simulink model "gnc_GlobalReplanner"  (R2026b)
settings: Solver=VariableStepAuto
values from neighbouring files (symbols this model uses):
  Ts = prm.Ts    [gnc_missionFSM.m]    (also in gnc_mpcPlantUpdate.m)
undefined symbols (not defined in the file or in its folder): P
settings Model: Creator=aomar  LastModifiedBy=aomar

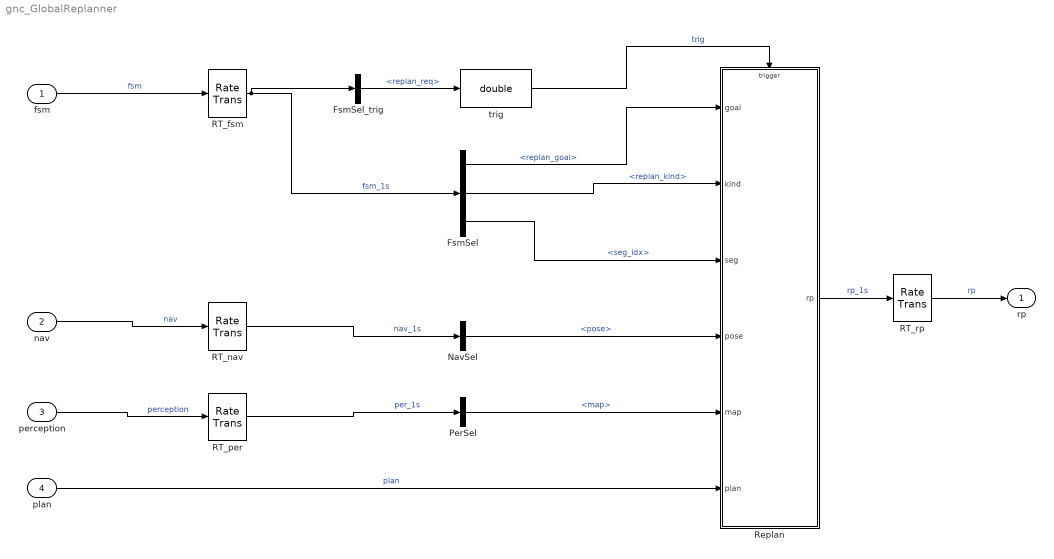
== system gnc_GlobalReplanner ==
  fsm : Inport  OutDataTypeStr=Bus: Bus_FsmOut  SampleTime=Ts.gnc
  nav : Inport  Port=2  OutDataTypeStr=Bus: Bus_NavCond  SampleTime=Ts.gnc
  perception : Inport  Port=3  OutDataTypeStr=Bus: Bus_Perception  SampleTime=Ts.perception
  plan : Inport  Port=4  OutDataTypeStr=Bus: Bus_MissionPlan
  FsmSel : BusSelector  OutputSignals=replan_goal,replan_kind,seg_idx
  FsmSel_trig : BusSelector  OutputSignals=replan_req
  NavSel : BusSelector  OutputSignals=pose
  PerSel : BusSelector  OutputSignals=map
  RT_fsm : RateTransition  OutPortSampleTime=Ts.plan
  RT_nav : RateTransition  OutPortSampleTime=Ts.plan
  RT_per : RateTransition  OutPortSampleTime=Ts.plan
  RT_rp : RateTransition  OutPortSampleTime=Ts.gnc
  Replan : Subsystem  TreatAsAtomicUnit=on
  trig : DataTypeConversion  OutDataTypeStr=double  RndMeth=Nearest
  rp : Outport  OutDataTypeStr=Bus: Bus_ReplanResult
  wires:
  fsm/1 -> RT_fsm/1  "fsm"
  nav/1 -> RT_nav/1  "nav"
  perception/1 -> RT_per/1  "perception"
  plan/1 -> Replan/6(plan)  "plan"
  RT_fsm/1 -> FsmSel/1, FsmSel_trig/1  "fsm_1s"
  RT_nav/1 -> NavSel/1  "nav_1s"
  RT_per/1 -> PerSel/1  "per_1s"
  FsmSel_trig/1 -> trig/1  "<replan_req>"
  FsmSel/1 -> Replan/1(goal)  "<replan_goal>"
  FsmSel/2 -> Replan/2(kind)  "<replan_kind>"
  FsmSel/3 -> Replan/3(seg)  "<seg_idx>"
  NavSel/1 -> Replan/4(pose)  "<pose>"
  PerSel/1 -> Replan/5(map)  "<map>"
  trig/1 -> Replan/Trigger  "trig"
  Replan/1(rp) -> RT_rp/1  "rp_1s"
  RT_rp/1 -> rp/1  "rp"

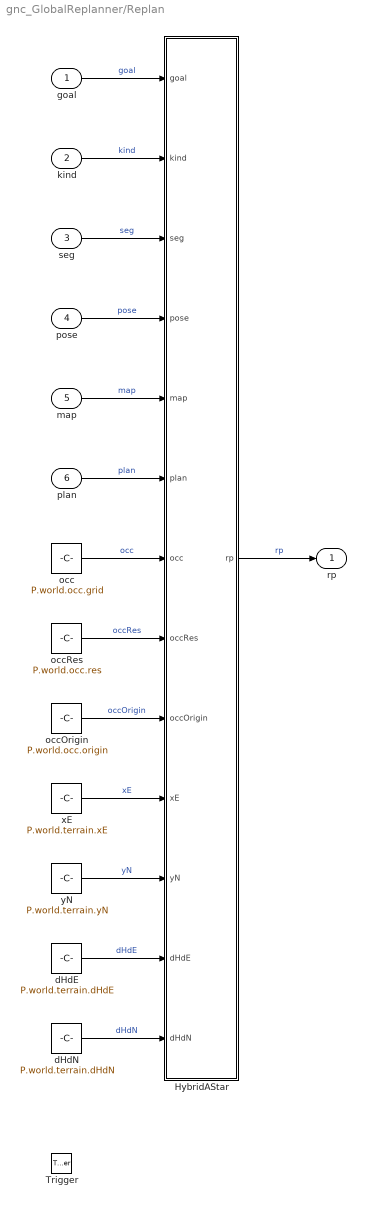
== system gnc_GlobalReplanner/Replan ==
  goal : Inport
  kind : Inport  Port=2
  seg : Inport  Port=3
  pose : Inport  Port=4
  map : Inport  Port=5
  plan : Inport  Port=6
  Trigger : TriggerPort  TriggerType=either  VariantControl=(inherit)  InitialTriggerSignalState=zero  PortDimensions=1
  HybridAStar : MATLAB Function  TreatAsAtomicUnit=on  mask{prm=P.gnc.hastar}
  dHdE : Constant  Value=P.world.terrain.dHdE  OutDataTypeStr=double
  dHdN : Constant  Value=P.world.terrain.dHdN  OutDataTypeStr=double
  occ : Constant  Value=P.world.occ.grid  OutDataTypeStr=boolean
  occOrigin : Constant  Value=P.world.occ.origin  OutDataTypeStr=double
  occRes : Constant  Value=P.world.occ.res  OutDataTypeStr=double
  xE : Constant  Value=P.world.terrain.xE  OutDataTypeStr=double
  yN : Constant  Value=P.world.terrain.yN  OutDataTypeStr=double
  rp : Outport  OutDataTypeStr=Bus: Bus_ReplanResult  InitialOutput=P.ic.Bus_ReplanResult
  wires:
  goal/1 -> HybridAStar/1(goal)  "goal"
  kind/1 -> HybridAStar/2(kind)  "kind"
  seg/1 -> HybridAStar/3(seg)  "seg"
  pose/1 -> HybridAStar/4(pose)  "pose"
  map/1 -> HybridAStar/5(map)  "map"
  plan/1 -> HybridAStar/6(plan)  "plan"
  occ/1 -> HybridAStar/7(occ)  "occ"
  occRes/1 -> HybridAStar/8(occRes)  "occRes"
  occOrigin/1 -> HybridAStar/9(occOrigin)  "occOrigin"
  xE/1 -> HybridAStar/10(xE)  "xE"
  yN/1 -> HybridAStar/11(yN)  "yN"
  dHdE/1 -> HybridAStar/12(dHdE)  "dHdE"
  dHdN/1 -> HybridAStar/13(dHdN)  "dHdN"
  HybridAStar/1(rp) -> rp/1  "rp"

== matlab function gnc_GlobalReplanner/Replan/HybridAStar ==
  settings: description=Hybrid A* replanning (gnc spec 4.4); body subsystems/gnc/gnc_globalReplanner.m.
  data: goal input; rp output Bus: Bus_ReplanResult; kind input; seg input; pose input; map input Bus: Bus_TebMapInfo; plan input Bus: Bus_MissionPlan; occ input; occRes input; occOrigin input; xE input; yN input; dHdE input; dHdN input; prm parameter
function rp = fcn(goal, kind, seg, pose, map, plan, occ, occRes, occOrigin, xE, yN, dHdE, dHdN, prm)
%#codegen
rp = gnc_globalReplanner(goal, kind, seg, pose, map, plan, occ, occRes, occOrigin, ...
    struct('xE', xE, 'yN', yN, 'dHdE', dHdE, 'dHdN', dHdN), prm);
